simulink model "a_test"  (R2022b)
settings: Solver=VariableStepAuto  StartTime=0.0  StopTime=10.0  RelTol=1e-3
values from neighbouring files (symbols this model uses):
  L = 0.00046    [electric_current_loop.m]    (also in electric_kp_ki.m; pll.m = 10000; sl_ekf.m = c.L_LINE; sl_flux.m = L_avg - 0.5 * L_diff + L_diff * iq_obs * iq_obs / i2_obs)
undefined symbols (not defined in the file or in its folder): D_PI_I, D_PI_KB, D_PI_LOW_LIMIT, D_PI_P, D_PI_UP_LIMIT, Q_PI_I, Q_PI_KB, Q_PI_LOW_LIMIT, Q_PI_P, Q_PI_UP_LIMIT
libraries: slpidlib x6, spsPermanentMagnetSynchronousMachineLib x4, simulink x4, spsDCVoltageSourceLib x2, spsGroundLib x2, spsThreePhaseVIMeasurementLib x2, spsUniversalBridgeLib x2, spspowerguiLib x2
(part 1 of 2)
settings Model: Creator=15403  LastModifiedBy=15403

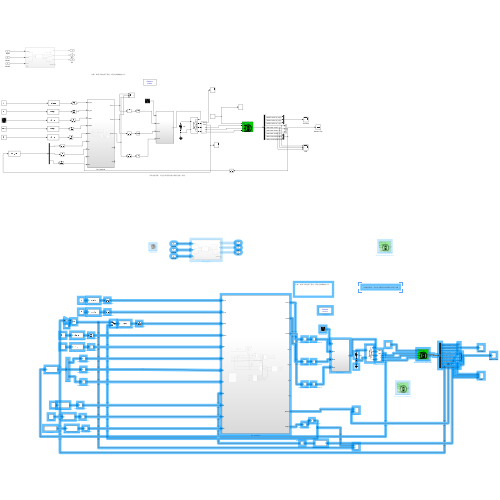
[thumbnail: Simulink's stored preview of the top-level diagram]
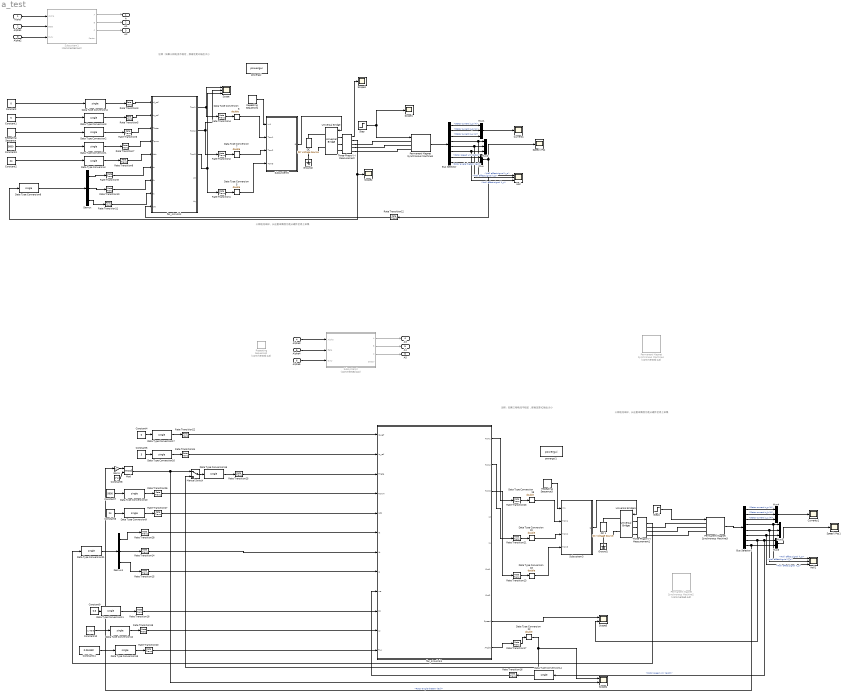
== system a_test ==
  note: 三相电流采样，从这里采集因为是从硬件全桥上采集
  note: 注释：如果三相电流不稳定，那肯定是IQ输出太小
  note: 注释：如果三相电流不稳定，那肯定是IQ输出太小
  note: 三相电流采样，从这里采集因为是从硬件全桥上采集
  Alpha : Inport
  Alpha1 : Inport  Port=2
  Alpha2 : Inport  Port=3
  Alpha3 : Inport  Port=4
  Alpha4 : Inport  Port=5
  Alpha5 : Inport  Port=6
  Bus Selector : BusSelector  OutputSignals=Stator current is_a (A),Stator current is_b (A),Stator current is_c (A),Hall effect signal h_a,Hall effect signal h_b,Hall effect signal h_c,Rotor speed wm (rad/s),Rotor angle thetam (rad)
  Bus Selector1 : BusSelector  OutputSignals=Stator current is_a (A),Stator current is_b (A),Stator current is_c (A),Hall effect signal h_a,Hall effect signal h_b,Hall effect signal h_c,Rotor speed wm (rad/s),Rotor angle thetam (rad)
  Constant : Constant  Value=0
  Constant1 : Constant  Value=5
  Constant10 : Constant  Value=1.4e-3
  Constant11 : Constant  Value=0.034182
  Constant2 : Constant  Value=24
  Constant3 : Constant  Value=5600
  Constant4 : Constant  Value=0
  Constant5 : Constant  Value=3
  Constant6 : Constant  Value=24
  Constant7 : Constant  Value=5600
  Constant8 : Constant  Value=2*pi
  Constant9 : Constant  Value=0.6
  Currents : Scope
  Currents1 : Scope
  "DC " : spsDCVoltageSourceLib/DC Voltage Source  Amplitude=24  Measurements=None
  DC 1 : spsDCVoltageSourceLib/DC Voltage Source  Amplitude=24  Measurements=None
  Data Type Conversion{,1..4,8..17,21} (16 alike) : DataTypeConversion  OutDataTypeStr=single  SaturateOnIntegerOverflow=off  RndMeth=Floor
  Data Type Conversion{5..7,18..20,22} (7 alike) : DataTypeConversion  OutDataTypeStr=double  SaturateOnIntegerOverflow=off  RndMeth=Floor
  Demux : Demux  Outputs=3
  Demux1 : Demux  Outputs=3
  Gain1 : Gain  OutDataTypeStr=double
  Ground1 : spsGroundLib/Ground  LConnTagsString=a
  Ground2 : spsGroundLib/Ground  LConnTagsString=a
  Hall : Scope  NumInputPorts=3
  Hall1 : Scope  NumInputPorts=3
  Manual Switch : ManualSwitch
  Mod : Math  Operator=mod  SignedPower=on
  Mux : Mux  Inputs=2
  Mux{1..2,4..5} (4 alike) : Mux  Inputs=3
  Mux3 : Mux  Inputs=2
  Permanent Magnet Synchronous Machine1 : spsPermanentMagnetSynchronousMachineLib/Permanent Magnet Synchronous Machine  NbPhases=3  FluxDistribution=Sinusoidal  RotorType=Round  MechanicalLoad=Torque Tm  PresetModel=No  ShowDetailedParameters=on  MeasurementBus=off  Resistance=0.6  Inductance=8.5e-3  dqInductances=[8.5e-3, 8.5e-3]  La=1.4e-3  MachineConstant=Flux linkage established by magnets (V.s)  Flux=0.034182  VoltageCst=6.1999  TorqueCst=0.051273  Flat=120  Mechanical=[1.1e-5,1e-4,1,0.02]  PolePairs=4  InitialConditions=[0,0, 0,0]  InitialConditions5ph=[0 0 0 0 0 0]  RefAngle=Aligned with phase A axis (original Park)  IterativeDiscreteModel=Trapezoidal non iterative  TsBlock=-1  TsPowergui=0
  Permanent Magnet Synchronous Machine2 : spsPermanentMagnetSynchronousMachineLib/Permanent Magnet Synchronous Machine  Commented=on  NbPhases=3  FluxDistribution=Sinusoidal  RotorType=Round  MechanicalLoad=Torque Tm  PresetModel=No  ShowDetailedParameters=on  MeasurementBus=off  Resistance=0.6  Inductance=8.5e-3  dqInductances=[8.5e-3, 8.5e-3]  La=1.4e-3  MachineConstant=Flux linkage established by magnets (V.s)  Flux=0.034182  VoltageCst=6.1999  TorqueCst=0.051273  Flat=120  Mechanical=[1.1e-5,1e-4,1,0.02]  PolePairs=4  InitialConditions=[0,0, 0,0]  InitialConditions5ph=[0 0 0 0 0 0]  RefAngle=Aligned with phase A axis (original Park)  IterativeDiscreteModel=Trapezoidal non iterative  TsBlock=-1  TsPowergui=0
  Permanent Magnet Synchronous Machine3 : spsPermanentMagnetSynchronousMachineLib/Permanent Magnet Synchronous Machine  NbPhases=3  FluxDistribution=Sinusoidal  RotorType=Round  MechanicalLoad=Torque Tm  PresetModel=No  ShowDetailedParameters=on  MeasurementBus=off  Resistance=0.6  Inductance=8.5e-3  dqInductances=[8.5e-3, 8.5e-3]  La=1.4e-3  MachineConstant=Flux linkage established by magnets (V.s)  Flux=0.034182  VoltageCst=6.1999  TorqueCst=0.051273  Flat=120  Mechanical=[1.1e-5,1e-4,1,0.02]  PolePairs=4  InitialConditions=[0,0, 0,0]  InitialConditions5ph=[0 0 0 0 0 0]  RefAngle=Aligned with phase A axis (original Park)  IterativeDiscreteModel=Trapezoidal non iterative  TsBlock=-1  TsPowergui=0
  Permanent Magnet Synchronous Machine4 : spsPermanentMagnetSynchronousMachineLib/Permanent Magnet Synchronous Machine  Commented=on  NbPhases=3  FluxDistribution=Sinusoidal  RotorType=Round  MechanicalLoad=Torque Tm  PresetModel=No  ShowDetailedParameters=on  MeasurementBus=off  Resistance=0.6  Inductance=8.5e-3  dqInductances=[8.5e-3, 8.5e-3]  La=1.4e-3  MachineConstant=Voltage Constant (V_peak L-L / krpm)  Flux=0.017643  VoltageCst=3.2  TorqueCst=0.026464  Flat=120  Mechanical=[1.1e-5,1e-4,1,0.02]  PolePairs=4  InitialConditions=[0,0, 0,0]  InitialConditions5ph=[0 0 0 0 0 0]  RefAngle=Aligned with phase A axis (original Park)  IterativeDiscreteModel=Trapezoidal non iterative  TsBlock=-1  TsPowergui=0
  Rate Transition{1..28} (28 alike) : RateTransition
  Repeating Sequence : simulink/Sources/Repeating Sequence  rep_seq_t=[0 0.1]  rep_seq_y=[0 2 * pi]
  Repeating Sequence1 : simulink/Sources/Repeating Sequence  rep_seq_t=[0 1/15000 2/15000]  rep_seq_y=[0 2800 0]
  Repeating Sequence2 : simulink/Sources/Repeating Sequence  Commented=on  rep_seq_t=[0 0.1]  rep_seq_y=[0 2 * pi]
  Repeating Sequence3 : simulink/Sources/Repeating Sequence  rep_seq_t=[0 1/15000 2/15000]  rep_seq_y=[0 2800 0]
  Scope : Scope  NumInputPorts=3
  Scope1 : Scope
  Scope2 : Scope
  Scope3 : Scope
  Scope4 : Scope  NumInputPorts=2
  Scope5 : Scope  NumInputPorts=2
  Speed / Pos : Scope
  Speed / Pos1 : Scope
  Step : Step  Time=0  After=0  SampleTime=0
  Step1 : Step  Time=0  After=0  SampleTime=0
  Subsystem1 : Subsystem  Commented=on
  Subsystem2 : Subsystem  Commented=on
  Subsystem3 : Subsystem
  Subsystem5 : Subsystem
  Three-Phase V-I Measurement : spsThreePhaseVIMeasurementLib/Three-Phase V-I Measurement  VoltageMeasurement=phase-to-ground  SetLabelV=off  LabelV=Vabc  Vpu=off  VpuLL=off  CurrentMeasurement=yes  SetLabelI=off  LabelI=Iabc  Ipu=off  Pbase=100e6  Vbase=500e3  OutputType=Complex  PhasorSimulation=off  PSBequivalent=0
  Three-Phase V-I Measurement1 : spsThreePhaseVIMeasurementLib/Three-Phase V-I Measurement  VoltageMeasurement=phase-to-ground  SetLabelV=off  LabelV=Vabc  Vpu=off  VpuLL=off  CurrentMeasurement=yes  SetLabelI=off  LabelI=Iabc  Ipu=off  Pbase=100e6  Vbase=500e3  OutputType=Complex  PhasorSimulation=off  PSBequivalent=0
  Universal Bridge : spsUniversalBridgeLib/Universal Bridge  Arms=3  SnubberResistance=1e5  SnubberCapacitance=inf  Device=IGBT / Diodes  Ron=1e-3  Lon=0  ForwardVoltages="[  0  0  ]"  ForwardVoltage=0  GTOparameters=[ 10e-6 , 20e-6 ]  IGBTparameters=[ 1e-6 , 2e-6 ]  Measurements=None  Measurements_2=None  converterType=Rectifier
  Universal Bridge1 : spsUniversalBridgeLib/Universal Bridge  Arms=3  SnubberResistance=1e5  SnubberCapacitance=inf  Device=IGBT / Diodes  Ron=1e-3  Lon=0  ForwardVoltages="[  0  0  ]"  ForwardVoltage=0  GTOparameters=[ 10e-6 , 20e-6 ]  IGBTparameters=[ 1e-6 , 2e-6 ]  Measurements=None  Measurements_2=None  converterType=Rectifier
  foc_simulink : Subsystem
  foc_simulink1 : Subsystem
  powergui : spspowerguiLib/powergui  Priority=1  SimulationMode=Discrete  SampleTime=0.000001  frequency=60  Iterations=50  frequencyindice=0  Pbase=100e6  ErrMax=1e-4  UnitsV=kV  UnitsW=MW  buscounter=0  FunctionMessages=off  echomessages=off  EnableUseOfTLC=off  CurrentSourceSwitches=off  DisableSnubberDevices=off  DisableRonSwitches=off  DisableVfSwitches=off  DisplayEquations=off  AutomaticDiscreteSolvers=off  SolverType=Tustin/Backward Euler (TBE)  Interpol=off  ExternalGateDelay=off  methode=off  Ts=100  x0status=blocks  SPID=on  SwTol=0  HookPort=off  NonlinearTolerance=1e-4  nMaxIteration=100  ContinueOnMaxIteration=off  RestoreLinks=warning  ResistiveCurrentMeasurement=off  Frange=[0:2:500]  Ylog=off  Xlog=on  ShowGrid=off  save=off  variable=ZData  structure=0  ZoomFFT=off  StartTime=0.0  cycles=1  DisplayStyle=1  fundamental=60  FreqAxis=off  MaxFrequency=1000  frequencyindicesteady=1  RmsSteady=1  display=off
  powergui1 : spspowerguiLib/powergui  Priority=1  SimulationMode=Discrete  SampleTime=0.000001  frequency=60  Iterations=50  frequencyindice=0  Pbase=100e6  ErrMax=1e-4  UnitsV=kV  UnitsW=MW  buscounter=0  FunctionMessages=off  echomessages=off  EnableUseOfTLC=off  CurrentSourceSwitches=off  DisableSnubberDevices=off  DisableRonSwitches=off  DisableVfSwitches=off  DisplayEquations=off  AutomaticDiscreteSolvers=off  SolverType=Tustin/Backward Euler (TBE)  Interpol=off  ExternalGateDelay=off  methode=off  Ts=100  x0status=blocks  SPID=on  SwTol=0  HookPort=off  NonlinearTolerance=1e-4  nMaxIteration=100  ContinueOnMaxIteration=off  RestoreLinks=warning  ResistiveCurrentMeasurement=off  Frange=[0:2:500]  Ylog=off  Xlog=on  ShowGrid=off  save=off  variable=ZData  structure=0  ZoomFFT=off  StartTime=0.0  cycles=1  DisplayStyle=1  fundamental=60  FreqAxis=off  MaxFrequency=1000  frequencyindicesteady=1  RmsSteady=1  display=off
  A : Outport
  A1 : Outport  Port=2
  A2 : Outport  Port=3
  A3 : Outport  Port=4
  A4 : Outport  Port=5
  A5 : Outport  Port=6
  wires:
  Data Type Conversion6/1 -> Subsystem5/2(Tcm1)
  Data Type Conversion8/1 -> Demux/1
  Rate Transition12/1 -> foc_simulink/9(we)
  Mux/1 -> Rate Transition12/1, Speed / Pos/1
  Three-Phase V-I Measurement/1 -> Scope3/1
  Demux/1 -> Rate Transition9/1
  Repeating Sequence/1 -> Data Type Conversion2/1
  Constant/1 -> Data Type Conversion4/1
  Alpha/1 -> Subsystem1/1(Alpha)
  Bus Selector/4 -> Hall/1, Mux2/1  "<Hall effect signal h_a>"
  Subsystem1/3(C) -> A2/1
  Data Type Conversion7/1 -> Subsystem5/3(Tcm2)
  Alpha2/1 -> Subsystem1/3(Duty)
  Data Type Conversion5/1 -> Subsystem5/4(Tcm3)
  Subsystem1/1(A) -> A/1
  Rate Transition6/1 -> foc_simulink/3(Theta)
  Data Type Conversion/1 -> Rate Transition8/1
  Rate Transition9/1 -> foc_simulink/6(Ia)
  Demux/2 -> Rate Transition10/1
  Rate Transition11/1 -> foc_simulink/8(Ic)
  Data Type Conversion1/1 -> Rate Transition7/1
  Subsystem1/2(B) -> A1/1
  Constant3/1 -> Data Type Conversion1/1
  Demux/3 -> Rate Transition11/1
  Rate Transition1/1 -> Data Type Conversion5/1
  Rate Transition10/1 -> foc_simulink/7(Ib)
  Repeating Sequence1/1 -> Subsystem5/1(In1)
  Subsystem5/1(g) -> Universal Bridge/1
  Rate Transition8/1 -> foc_simulink/5(Udc)
  Rate Transition4/1 -> Data Type Conversion6/1
  Rate Transition5/1 -> foc_simulink/2(Iq_ref)
  Constant1/1 -> Data Type Conversion3/1
  Rate Transition2/1 -> Data Type Conversion7/1
  Permanent Magnet Synchronous Machine1/1 -> Bus Selector/1
  Data Type Conversion2/1 -> Rate Transition6/1
  Step/1 -> Permanent Magnet Synchronous Machine1/1, Scope1/1
  Mux1/1 -> Currents/1
  Bus Selector/6 -> Mux2/3, Hall/3  "<Hall effect signal h_c>"
  Bus Selector/1 -> Mux1/1  "<Stator current is_a (A)>"
  Rate Transition3/1 -> foc_simulink/1(Id_ref)
  Data Type Conversion3/1 -> Rate Transition5/1
  Bus Selector/3 -> Mux1/3  "<Stator current is_c (A)>"
  Constant2/1 -> Data Type Conversion/1
  Bus Selector/8 -> Mux/2  "<Rotor angle thetam (rad)>"
  Bus Selector/5 -> Mux2/2, Hall/2  "<Hall effect signal h_b>"
  Rate Transition7/1 -> foc_simulink/4(Tpwm)
  foc_simulink/2(Tcm2) -> Rate Transition2/1, Scope/2
  Three-Phase V-I Measurement/2 -> Scope2/1, Data Type Conversion8/1
  Data Type Conversion4/1 -> Rate Transition3/1
  foc_simulink/1(Tcm1) -> Rate Transition4/1, Scope/1
  Bus Selector/7 -> Mux/1  "<Rotor speed wm (rad/s)>"
  foc_simulink/3(Tcm3) -> Rate Transition1/1, Scope/3
  Bus Selector/2 -> Mux1/2  "<Stator current is_b (A)>"
  Alpha1/1 -> Subsystem1/2(Beta)
  Data Type Conversion14/1 -> Rate Transition16/1
  Mod/1 -> Scope4/2, Manual Switch/1
  Data Type Conversion18/1 -> Subsystem3/4(Tcm3)
  foc_simulink1/8(Speed) -> Scope5/1
  foc_simulink1/3(Tcm3) -> Rate Transition13/1
  Permanent Magnet Synchronous Machine3/1 -> Bus Selector1/1
  foc_simulink1/9(Angle) -> Rate Transition17/1
  Rate Transition19/1 -> foc_simulink1/11(Ls)
  Constant11/1 -> Data Type Conversion13/1
  Data Type Conversion13/1 -> Rate Transition20/1
  Gain1/1 -> Mod/1
  Rate Transition28/1 -> foc_simulink1/6(Ia)
  Alpha4/1 -> Subsystem2/2(Beta)
  Rate Transition18/1 -> foc_simulink1/10(Rs)
  Data Type Conversion16/1 -> Rate Transition24/1
  Rate Transition21/1 -> Data Type Conversion20/1
  Rate Transition20/1 -> foc_simulink1/12(flux)
  Bus Selector1/7 -> Scope5/2, Data Type Conversion14/1, Mux3/1  "<Rotor speed wm (rad/s)>"
  Bus Selector1/5 -> Mux5/2, Hall1/2  "<Hall effect signal h_b>"
  Subsystem2/3(C) -> A5/1
  Data Type Conversion15/1 -> Rate Transition25/1
  Bus Selector1/2 -> Mux4/2  "<Stator current is_b (A)>"
  Data Type Conversion11/1 -> Rate Transition18/1
  Manual Switch/1 -> Data Type Conversion15/1
  Step1/1 -> Permanent Magnet Synchronous Machine3/1
  Subsystem3/1(g) -> Universal Bridge1/1
  Bus Selector1/3 -> Mux4/3  "<Stator current is_c (A)>"
  Data Type Conversion22/1 -> Scope4/1, Manual Switch/2
  Three-Phase V-I Measurement1/2 -> Data Type Conversion21/1
  foc_simulink1/1(Tcm1) -> Rate Transition23/1
  foc_simulink1/2(Tcm2) -> Rate Transition21/1
  Rate Transition26/1 -> foc_simulink1/4(Tpwm)
  Constant9/1 -> Data Type Conversion11/1
  Constant5/1 -> Data Type Conversion16/1
  Bus Selector1/6 -> Mux5/3, Hall1/3  "<Hall effect signal h_c>"
  Constant8/1 -> Mod/2
  Constant6/1 -> Data Type Conversion9/1
  Bus Selector1/8 -> Mux3/2, Gain1/1  "<Rotor angle thetam (rad)>"
  Bus Selector1/1 -> Mux4/1  "<Stator current is_a (A)>"
  Rate Transition27/1 -> foc_simulink1/5(Udc)
  Subsystem2/1(A) -> A3/1
  Rate Transition22/1 -> foc_simulink1/1(Id_ref)
  Bus Selector1/4 -> Hall1/1, Mux5/1  "<Hall effect signal h_a>"
  Mux4/1 -> Currents1/1
  Demux1/1 -> Rate Transition28/1
  Data Type Conversion21/1 -> Demux1/1
  Rate Transition24/1 -> foc_simulink1/2(Iq_ref)
  Repeating Sequence3/1 -> Subsystem3/1(In1)
  Rate Transition25/1 -> foc_simulink1/3(Theta)
  Alpha3/1 -> Subsystem2/1(Alpha)
  Demux1/3 -> Rate Transition15/1
  Demux1/2 -> Rate Transition14/1
  Data Type Conversion20/1 -> Subsystem3/3(Tcm2)
  Constant4/1 -> Data Type Conversion17/1
  Constant7/1 -> Data Type Conversion10/1
  Rate Transition13/1 -> Data Type Conversion18/1
  Mux3/1 -> Speed / Pos1/1
  Constant10/1 -> Data Type Conversion12/1
  Subsystem2/2(B) -> A4/1
  Rate Transition17/1 -> Data Type Conversion22/1
  Rate Transition15/1 -> foc_simulink1/8(Ic)
  Data Type Conversion17/1 -> Rate Transition22/1
  Data Type Conversion10/1 -> Rate Transition26/1
  Data Type Conversion9/1 -> Rate Transition27/1
  Alpha5/1 -> Subsystem2/3(Duty)
  Rate Transition14/1 -> foc_simulink1/7(Ib)
  Data Type Conversion12/1 -> Rate Transition19/1
  Rate Transition23/1 -> Data Type Conversion19/1
  Rate Transition16/1 -> foc_simulink1/9(we)
  Data Type Conversion19/1 -> Subsystem3/2(Tcm1)
  connections:
  Ground2/LConn1 -- "DC "/LConn1 -- Universal Bridge/RConn2
  "DC "/RConn1 -- Universal Bridge/RConn1
  Universal Bridge/LConn2 -- Three-Phase V-I Measurement/LConn2
  Three-Phase V-I Measurement/RConn3 -- Permanent Magnet Synchronous Machine1/LConn3
  Universal Bridge/LConn3 -- Three-Phase V-I Measurement/LConn3
  Three-Phase V-I Measurement/RConn2 -- Permanent Magnet Synchronous Machine1/LConn2
  Universal Bridge/LConn1 -- Three-Phase V-I Measurement/LConn1
  Three-Phase V-I Measurement/RConn1 -- Permanent Magnet Synchronous Machine1/LConn1
  Universal Bridge1/RConn2 -- Ground1/LConn1 -- DC 1/LConn1
  Universal Bridge1/LConn2 -- Three-Phase V-I Measurement1/LConn2
  Permanent Magnet Synchronous Machine3/LConn2 -- Three-Phase V-I Measurement1/RConn2
  Universal Bridge1/LConn1 -- Three-Phase V-I Measurement1/LConn1
  DC 1/RConn1 -- Universal Bridge1/RConn1
  Universal Bridge1/LConn3 -- Three-Phase V-I Measurement1/LConn3
  Permanent Magnet Synchronous Machine3/LConn3 -- Three-Phase V-I Measurement1/RConn3
  Permanent Magnet Synchronous Machine3/LConn1 -- Three-Phase V-I Measurement1/RConn1

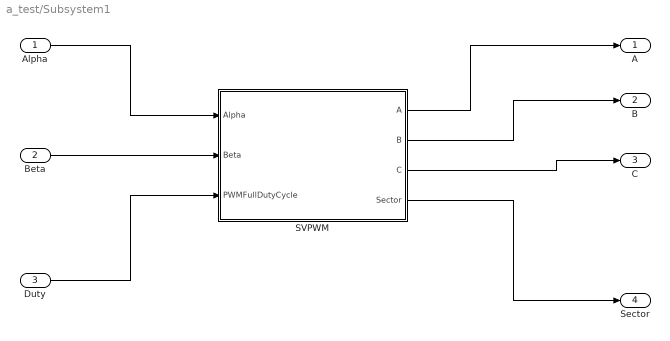
== system a_test/Subsystem1 ==
  Alpha : Inport
  Beta : Inport  Port=2
  Duty : Inport  Port=3
  SVPWM : MATLAB Function  TreatAsAtomicUnit=on
  A : Outport
  B : Outport  Port=2
  C : Outport  Port=3
  Sector : Outport  Port=4
  wires:
  SVPWM/1(A) -> A/1
  Duty/1 -> SVPWM/3(PWMFullDutyCycle)
  Alpha/1 -> SVPWM/1(Alpha)
  Beta/1 -> SVPWM/2(Beta)
  SVPWM/3(C) -> C/1
  SVPWM/4(Sector) -> Sector/1
  SVPWM/2(B) -> B/1

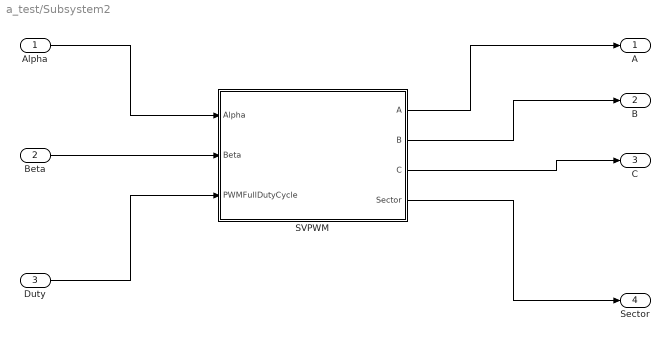
== system a_test/Subsystem2 ==
  Alpha : Inport
  Beta : Inport  Port=2
  Duty : Inport  Port=3
  SVPWM : MATLAB Function  TreatAsAtomicUnit=on
  A : Outport
  B : Outport  Port=2
  C : Outport  Port=3
  Sector : Outport  Port=4
  wires:
  SVPWM/1(A) -> A/1
  Duty/1 -> SVPWM/3(PWMFullDutyCycle)
  Alpha/1 -> SVPWM/1(Alpha)
  Beta/1 -> SVPWM/2(Beta)
  SVPWM/3(C) -> C/1
  SVPWM/4(Sector) -> Sector/1
  SVPWM/2(B) -> B/1

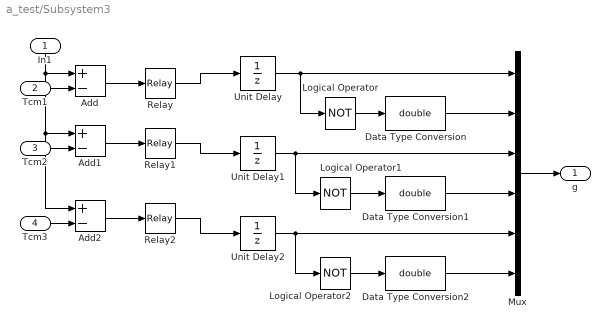
== system a_test/Subsystem3 ==
  In1 : Inport
  Tcm1 : Inport  Port=2
  Tcm2 : Inport  Port=3
  Tcm3 : Inport  Port=4
  Add : Sum  Inputs=+-
  Add1 : Sum  Inputs=+-
  Add2 : Sum  Inputs=+-
  Data Type Conversion : DataTypeConversion  OutDataTypeStr=double  SaturateOnIntegerOverflow=off  RndMeth=Floor
  Data Type Conversion1 : DataTypeConversion  OutDataTypeStr=double  SaturateOnIntegerOverflow=off  RndMeth=Floor
  Data Type Conversion2 : DataTypeConversion  OutDataTypeStr=double  SaturateOnIntegerOverflow=off  RndMeth=Floor
  Logical Operator : Logic  Operator=NOT  AllPortsSameDT=off  OutDataTypeStr=boolean
  Logical Operator1 : Logic  Operator=NOT  AllPortsSameDT=off  OutDataTypeStr=boolean
  Logical Operator2 : Logic  Operator=NOT  AllPortsSameDT=off  OutDataTypeStr=boolean
  Mux : Mux  Inputs=6
  Relay : Relay  OffSwitchValue=-eps
  Relay1 : Relay  OffSwitchValue=-eps
  Relay2 : Relay  OffSwitchValue=-eps
  Unit Delay : UnitDelay  SampleTime=-1  HasFrameUpgradeWarning=on
  Unit Delay1 : UnitDelay  SampleTime=-1  HasFrameUpgradeWarning=on
  Unit Delay2 : UnitDelay  SampleTime=-1  HasFrameUpgradeWarning=on
  g : Outport  VectorParamsAs1DForOutWhenUnconnected=off
  wires:
  Tcm3/1 -> Add2/2
  Tcm2/1 -> Add1/2
  Tcm1/1 -> Add/2
  Relay2/1 -> Unit Delay2/1
  Relay1/1 -> Unit Delay1/1
  Relay/1 -> Unit Delay/1
  Unit Delay2/1 -> Mux/5, Logical Operator2/1
  Unit Delay1/1 -> Mux/3, Logical Operator1/1
  Unit Delay/1 -> Logical Operator/1, Mux/1
  Mux/1 -> g/1
  Data Type Conversion/1 -> Mux/2
  Data Type Conversion1/1 -> Mux/4
  Data Type Conversion2/1 -> Mux/6
  Logical Operator2/1 -> Data Type Conversion2/1
  Logical Operator1/1 -> Data Type Conversion1/1
  Logical Operator/1 -> Data Type Conversion/1
  Add1/1 -> Relay1/1
  Add2/1 -> Relay2/1
  Add/1 -> Relay/1
  In1/1 -> Add/1, Add2/1, Add1/1

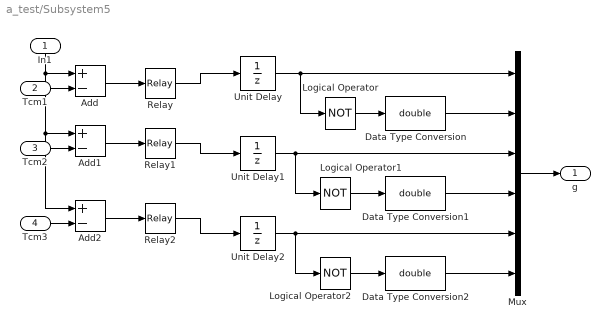
== system a_test/Subsystem5 ==
  In1 : Inport
  Tcm1 : Inport  Port=2
  Tcm2 : Inport  Port=3
  Tcm3 : Inport  Port=4
  Add : Sum  Inputs=+-
  Add1 : Sum  Inputs=+-
  Add2 : Sum  Inputs=+-
  Data Type Conversion : DataTypeConversion  OutDataTypeStr=double  SaturateOnIntegerOverflow=off  RndMeth=Floor
  Data Type Conversion1 : DataTypeConversion  OutDataTypeStr=double  SaturateOnIntegerOverflow=off  RndMeth=Floor
  Data Type Conversion2 : DataTypeConversion  OutDataTypeStr=double  SaturateOnIntegerOverflow=off  RndMeth=Floor
  Logical Operator : Logic  Operator=NOT  AllPortsSameDT=off  OutDataTypeStr=boolean
  Logical Operator1 : Logic  Operator=NOT  AllPortsSameDT=off  OutDataTypeStr=boolean
  Logical Operator2 : Logic  Operator=NOT  AllPortsSameDT=off  OutDataTypeStr=boolean
  Mux : Mux  Inputs=6
  Relay : Relay  OffSwitchValue=-eps
  Relay1 : Relay  OffSwitchValue=-eps
  Relay2 : Relay  OffSwitchValue=-eps
  Unit Delay : UnitDelay  SampleTime=-1  HasFrameUpgradeWarning=on
  Unit Delay1 : UnitDelay  SampleTime=-1  HasFrameUpgradeWarning=on
  Unit Delay2 : UnitDelay  SampleTime=-1  HasFrameUpgradeWarning=on
  g : Outport  VectorParamsAs1DForOutWhenUnconnected=off
  wires:
  Tcm3/1 -> Add2/2
  Tcm2/1 -> Add1/2
  Tcm1/1 -> Add/2
  Relay2/1 -> Unit Delay2/1
  Relay1/1 -> Unit Delay1/1
  Relay/1 -> Unit Delay/1
  Unit Delay2/1 -> Mux/5, Logical Operator2/1
  Unit Delay1/1 -> Mux/3, Logical Operator1/1
  Unit Delay/1 -> Logical Operator/1, Mux/1
  Mux/1 -> g/1
  Data Type Conversion/1 -> Mux/2
  Data Type Conversion1/1 -> Mux/4
  Data Type Conversion2/1 -> Mux/6
  Logical Operator2/1 -> Data Type Conversion2/1
  Logical Operator1/1 -> Data Type Conversion1/1
  Logical Operator/1 -> Data Type Conversion/1
  Add1/1 -> Relay1/1
  Add2/1 -> Relay2/1
  Add/1 -> Relay/1
  In1/1 -> Add/1, Add2/1, Add1/1

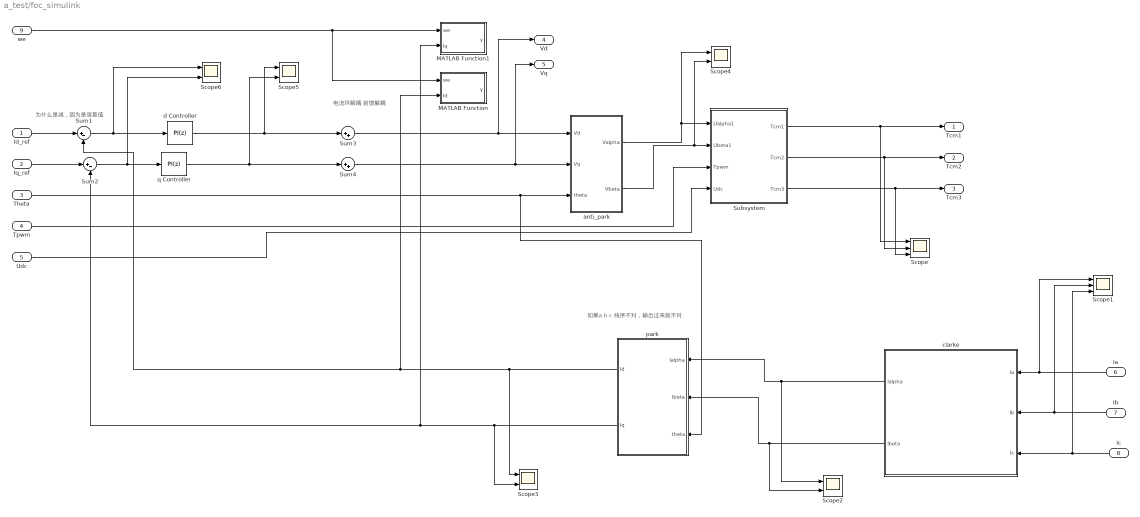
== system a_test/foc_simulink ==
  note: 电流环解耦
      | 前馈解耦
  note: 为什么是减，因为是误差值
  note: 如果a b c 线序不对，输出过来就不对
  Id_ref : Inport
  Iq_ref : Inport  Port=2
  Theta : Inport  Port=3
  Tpwm : Inport  Port=4
  Udc : Inport  Port=5
  Ia : Inport  Port=6
  Ib : Inport  Port=7
  Ic : Inport  Port=8
  we : Inport  Port=9
  MATLAB Function : MATLAB Function  TreatAsAtomicUnit=on
  MATLAB Function1 : MATLAB Function  TreatAsAtomicUnit=on
  Scope : Scope  NumInputPorts=3
  Scope1 : Scope  NumInputPorts=3
  Scope{2..6} (5 alike) : Scope  NumInputPorts=2
  Subsystem : Subsystem
  Sum1 : Sum  Inputs=|+-
  Sum2 : Sum  Inputs=|+-
  Sum3 : Sum  Inputs=|++  AccumDataTypeStr=single  OutDataTypeStr=single
  Sum4 : Sum  Inputs=|++  AccumDataTypeStr=single  OutDataTypeStr=single
  anti_park : Subsystem
  clarke : Subsystem
  d Controller : slpidlib/PID Controller  Controller=PI  Form=Parallel  TimeDomain=Discrete-time  UseExternalTs=off  SampleTime=-1  IntegratorMethod=Forward Euler  FilterMethod=Forward Euler  ControllerParametersSource=internal  P=D_PI_P  I=D_PI_I  UseKiTs=off  D=0.09  N=100  UseFilter=on  TunerSelectOption=Transfer Function Based (PID Tuner App)  InitialConditionSource=internal  InitialConditionForIntegrator=0  InitialConditionForFilter=0  DifferentiatorICPrevScaledInput=0  ExternalReset=none  TrackingMode=off  Kt=1  LimitOutput=on  SatLimitsSource=internal  UpperSaturationLimit=D_PI_UP_LIMIT  LowerSaturationLimit=D_PI_LOW_LIMIT  LinearizeAsGain=off  AntiWindupMode=back-calculation  Kb=D_PI_KB  LimitIntegrator=off  UpperIntegratorSaturationLimit=inf  LowerIntegratorSaturationLimit=-inf  PGainOutDataTypeStr=single  PProdOutDataTypeStr=single  POutMin=[]  POutMax=[]  IGainOutDataTypeStr=single  IProdOutDataTypeStr=single  IOutMin=[]  IOutMax=[]  DOutMin=[]  DOutMax=[]  NOutMin=[]  NOutMax=[]  SumOutDataTypeStr=single  SumOutMin=[]  SumOutMax=[]  SaturationOutDataTypeStr=single  SaturationOutMin=[]  SaturationOutMax=[]  PParamDataTypeStr=single  PParamMin=[]  PParamMax=[]  IParamDataTypeStr=single  IParamMin=[]  IParamMax=[]  DParamMin=[]  DParamMax=[]  NParamMin=[]  NParamMax=[]  KbParamDataTypeStr=single  KbParamMin=[]  KbParamMax=[]  KtParamMin=[]  KtParamMax=[]  KbOutDataTypeStr=single  KbOutMin=[]  KbOutMax=[]  KtOutMin=[]  KtOutMax=[]  IntegratorOutDataTypeStr=single  IntegratorOutMin=[]  IntegratorOutMax=[]  FilterOutMin=[]  FilterOutMax=[]  SumI1OutDataTypeStr=single  SumI1OutMin=[]  SumI1OutMax=[]  SumI2OutDataTypeStr=single  SumI2OutMin=[]  SumI2OutMax=[]  SumI3OutMin=[]  SumI3OutMax=[]  SumI4OutMin=[]  SumI4OutMax=[]  SumDOutMin=[]  SumDOutMax=[]  SumAccumDataTypeStr=single  SumI1AccumDataTypeStr=single  SumI2AccumDataTypeStr=single  DifferentiatorOutMin=[]  DifferentiatorOutMax=[]  FilterDiffOutCoefMin=[]  FilterDiffOutCoefMax=[]  ReciprocalOutMin=[]  ReciprocalOutMax=[]  SumDenOutMin=[]  SumDenOutMax=[]  SumNumOutMin=[]  SumNumOutMax=[]  DivideOutMin=[]  DivideOutMax=[]  UdiffTsProdOutMin=[]  UdiffTsProdOutMax=[]  NTsProdOutMin=[]  NTsProdOutMax=[]  UintegralTsProdOutMin=[]  UintegralTsProdOutMax=[]  UngainTsProdOutMin=[]  UngainTsProdOutMax=[]  ClampingZeroOutDataTypeStr=Inherit: Inherit via back propagation  ClampingZeroOutMin=[]  ClampingZeroOutMax=[]  FilterDenConstantOutDataTypeStr=Inherit: Inherit via back propagation  FilterDenConstantOutMin=[]  FilterDenConstantOutMax=[]  PCopyOutDataTypeStr=Inherit: Inherit via back propagation  PCopyOutMin=[]  PCopyOutMax=[]  NCopyOutDataTypeStr=Inherit: Inherit via back propagation  NCopyOutMin=[]  NCopyOutMax=[]  IntegratorContinuousStateAttributes=''  IntegratorStateIdentifier=di  IntegratorStateMustResolveToSignalObject=off  IntegratorRTWStateStorageClass=Auto  FilterContinuousStateAttributes=''  FilterStateMustResolveToSignalObject=off  FilterRTWStateStorageClass=Auto  ParallelPVariant=InternalParameters  IdealPVariant=Disabled  IVariant=InternalParameters  DVariant=Disabled  IntegratorVariant=Discrete  SatVariant=Enabled  AWVariant=BackCalculation  PCopyVariant=Disabled  TRVariant=Disabled  FdbkBlocksVariant=Forward  IdealPFdbkVariant=Disabled  SatFdbkVariant=Disabled  DerivativeFilterVariant=Disabled  NVariant=Disabled  NCopyVariant=Disabled_SignalSpec  FilterICVariant=Disabled  IntegratorICVariant=InternalICs  ExternalResetVariant=Disabled  TRSumVariant=Passthrough  SumFdbkVariant=Disabled  SumVariant=Sum_PI  TsampFilterVariant=InternalTs  TsampNgainVariant=Passthrough  TsampIntegralVariant=Passthrough  ExternalSaturationOutDataTypeStr=Inherit: Same as second input
  park : Subsystem
  q Controller : slpidlib/PID Controller  Controller=PI  Form=Parallel  TimeDomain=Discrete-time  UseExternalTs=off  SampleTime=-1  IntegratorMethod=Forward Euler  FilterMethod=Forward Euler  ControllerParametersSource=internal  P=Q_PI_P  I=Q_PI_I  UseKiTs=off  D=0.09  N=100  UseFilter=on  TunerSelectOption=Transfer Function Based (PID Tuner App)  InitialConditionSource=internal  InitialConditionForIntegrator=0  InitialConditionForFilter=0  DifferentiatorICPrevScaledInput=0  ExternalReset=none  TrackingMode=off  Kt=1  LimitOutput=on  SatLimitsSource=internal  UpperSaturationLimit=Q_PI_UP_LIMIT  LowerSaturationLimit=Q_PI_LOW_LIMIT  LinearizeAsGain=off  AntiWindupMode=back-calculation  Kb=Q_PI_KB  LimitIntegrator=off  UpperIntegratorSaturationLimit=inf  LowerIntegratorSaturationLimit=-inf  PGainOutDataTypeStr=single  PProdOutDataTypeStr=single  POutMin=[]  POutMax=[]  IGainOutDataTypeStr=single  IProdOutDataTypeStr=single  IOutMin=[]  IOutMax=[]  DOutMin=[]  DOutMax=[]  NOutMin=[]  NOutMax=[]  SumOutDataTypeStr=single  SumOutMin=[]  SumOutMax=[]  SaturationOutDataTypeStr=single  SaturationOutMin=[]  SaturationOutMax=[]  PParamDataTypeStr=single  PParamMin=[]  PParamMax=[]  IParamDataTypeStr=single  IParamMin=[]  IParamMax=[]  DParamMin=[]  DParamMax=[]  NParamMin=[]  NParamMax=[]  KbParamDataTypeStr=single  KbParamMin=[]  KbParamMax=[]  KtParamMin=[]  KtParamMax=[]  KbOutDataTypeStr=single  KbOutMin=[]  KbOutMax=[]  KtOutMin=[]  KtOutMax=[]  IntegratorOutDataTypeStr=single  IntegratorOutMin=[]  IntegratorOutMax=[]  FilterOutMin=[]  FilterOutMax=[]  SumI1OutDataTypeStr=single  SumI1OutMin=[]  SumI1OutMax=[]  SumI2OutDataTypeStr=single  SumI2OutMin=[]  SumI2OutMax=[]  SumI3OutMin=[]  SumI3OutMax=[]  SumI4OutMin=[]  SumI4OutMax=[]  SumDOutMin=[]  SumDOutMax=[]  SumAccumDataTypeStr=single  SumI1AccumDataTypeStr=single  SumI2AccumDataTypeStr=single  DifferentiatorOutMin=[]  DifferentiatorOutMax=[]  FilterDiffOutCoefMin=[]  FilterDiffOutCoefMax=[]  ReciprocalOutMin=[]  ReciprocalOutMax=[]  SumDenOutMin=[]  SumDenOutMax=[]  SumNumOutMin=[]  SumNumOutMax=[]  DivideOutMin=[]  DivideOutMax=[]  UdiffTsProdOutMin=[]  UdiffTsProdOutMax=[]  NTsProdOutMin=[]  NTsProdOutMax=[]  UintegralTsProdOutMin=[]  UintegralTsProdOutMax=[]  UngainTsProdOutMin=[]  UngainTsProdOutMax=[]  ClampingZeroOutDataTypeStr=Inherit: Inherit via back propagation  ClampingZeroOutMin=[]  ClampingZeroOutMax=[]  FilterDenConstantOutDataTypeStr=Inherit: Inherit via back propagation  FilterDenConstantOutMin=[]  FilterDenConstantOutMax=[]  PCopyOutDataTypeStr=Inherit: Inherit via back propagation  PCopyOutMin=[]  PCopyOutMax=[]  NCopyOutDataTypeStr=Inherit: Inherit via back propagation  NCopyOutMin=[]  NCopyOutMax=[]  IntegratorContinuousStateAttributes=''  IntegratorStateIdentifier=qi  IntegratorStateMustResolveToSignalObject=off  IntegratorRTWStateStorageClass=Auto  FilterContinuousStateAttributes=''  FilterStateMustResolveToSignalObject=off  FilterRTWStateStorageClass=Auto  ParallelPVariant=InternalParameters  IdealPVariant=Disabled  IVariant=InternalParameters  DVariant=Disabled  IntegratorVariant=Discrete  SatVariant=Enabled  AWVariant=BackCalculation  PCopyVariant=Disabled  TRVariant=Disabled  FdbkBlocksVariant=Forward  IdealPFdbkVariant=Disabled  SatFdbkVariant=Disabled  DerivativeFilterVariant=Disabled  NVariant=Disabled  NCopyVariant=Disabled_SignalSpec  FilterICVariant=Disabled  IntegratorICVariant=InternalICs  ExternalResetVariant=Disabled  TRSumVariant=Passthrough  SumFdbkVariant=Disabled  SumVariant=Sum_PI  TsampFilterVariant=InternalTs  TsampNgainVariant=Passthrough  TsampIntegralVariant=Passthrough  ExternalSaturationOutDataTypeStr=Inherit: Same as second input
  Tcm1 : Outport
  Tcm2 : Outport  Port=2
  Tcm3 : Outport  Port=3
  Vd : Outport  Port=4
  Vq : Outport  Port=5
  wires:
  Theta/1 -> anti_park/3(theta), park/3(theta)
  Udc/1 -> Subsystem/4(Udc)
  Tpwm/1 -> Subsystem/3(Tpwm)
  Subsystem/3(Tcm3) -> Scope/3, Tcm3/1
  anti_park/2(Vbeta) -> Scope4/2, Subsystem/2(Ubeta1)
  Subsystem/1(Tcm1) -> Scope/1, Tcm1/1
  Subsystem/2(Tcm2) -> Scope/2, Tcm2/1
  anti_park/1(Valpha) -> Scope4/1, Subsystem/1(Ualpha1)
  clarke/2(Ibeta) -> Scope2/2, park/2(Ibeta)
  clarke/1(Ialpha) -> Scope2/1, park/1(Ialpha)
  Ia/1 -> Scope1/1, clarke/1(Ia)
  Ib/1 -> Scope1/2, clarke/2(Ib)
  Ic/1 -> Scope1/3, clarke/3(Ic)
  park/1(Id) -> MATLAB Function/2(Id), Sum1/2, Scope3/1
  park/2(Iq) -> Scope3/2, Sum2/2, MATLAB Function1/2(Iq)
  Id_ref/1 -> Sum1/1
  Sum1/1 -> Scope6/1, d Controller/1
  Iq_ref/1 -> Sum2/1
  Sum2/1 -> Scope6/2, q Controller/1
  d Controller/1 -> Scope5/1, Sum3/1
  q Controller/1 -> Scope5/2, Sum4/1
  we/1 -> MATLAB Function/1(we), MATLAB Function1/1(we)
  Sum4/1 -> Vq/1, anti_park/2(Vq)
  Sum3/1 -> Vd/1, anti_park/1(Vd)

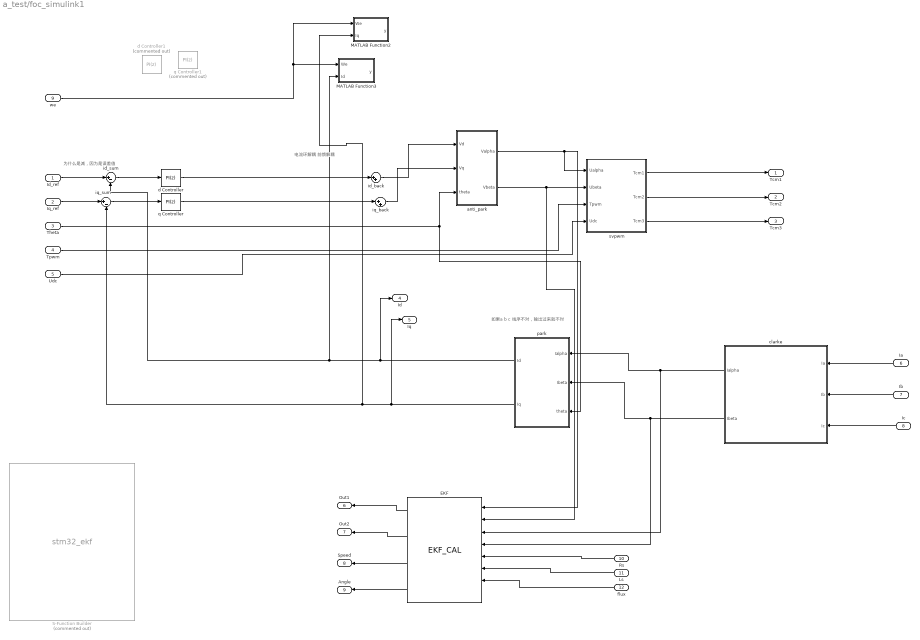
== system a_test/foc_simulink1 ==
  note: 电流环解耦
      | 前馈解耦
  note: 为什么是减，因为是误差值
  note: 如果a b c 线序不对，输出过来就不对
  Id_ref : Inport
  Iq_ref : Inport  Port=2
  Theta : Inport  Port=3
  Tpwm : Inport  Port=4
  Udc : Inport  Port=5
  Ia : Inport  Port=6
  Ib : Inport  Port=7
  Ic : Inport  Port=8
  we : Inport  Port=9
  Rs : Inport  Port=10
  Ls : Inport  Port=11
  flux : Inport  Port=12
  EKF : S-Function  FunctionName=EKF_CAL  SFunctionDeploymentMode=off  EnableBusSupport=off  mask(S-Function Builder){}
      mask help: Simulink:masks:SFunctionBuilder_MD
      mask init:
      | val = [[.9  0.75 0.75 1 1 .9 .9 1]',[1 1 0.75 0.75 .9 .9 1 .9]'];try , sys = get_param(gcb,'SfunBuilderFcnName');if isempty(sys), sys = get_param(gcb,'FunctionName'); end,catch, sys = get_param(gcb,'FunctionName'); end
      settings: CopyFcn=set_param(gcbh,'LinkStatus','none')  OpenFcn=sfunctionwizard(gcbh)
      mask Display: plot(val(:,1),val(:,2)),disp(sys),port_label('input',1,'Ualpha'),port_label('input',2,'Ubeta'),port_label('input',3,'Ialpha'),port_label('input',4,'Ibeta'),port_label('input',5,'Rs_in'),port_label('input',6,'Flux_in'),port_label('input',7,'Ls_in'),port_label('output',1,'y0'),port_label('output',2,'y1'),port_label('output',3,'Speed'),port_label('output',4,'Angle')
  MATLAB Function2 : MATLAB Function  TreatAsAtomicUnit=on
  MATLAB Function3 : MATLAB Function  TreatAsAtomicUnit=on
  S-Function Builder : S-Function  Commented=on  InitFcn=try, set_param(gcb,'FunctionName','stm32_ekf'), end  FunctionName=stm32_ekf  SFunctionModules=stm32_ekf_wrapper  SFunctionDeploymentMode=off  EnableBusSupport=off  mask(S-Function Builder){}
      mask help: Simulink:masks:SFunctionBuilder_MD
      mask init: same as a_test/foc_simulink1/EKF
      settings: CopyFcn=set_param(gcbh,'LinkStatus','none')  PreSaveFcn=try, set_param(gcb,'FunctionName','stm32_ekf'), end  OpenFcn=sfunctionwizard(gcbh)
      mask Display: plot(val(:,1),val(:,2)),disp(sys),port_label('input',1,'Ualpha'),port_label('input',2,'Ubeta'),port_label('input',3,'Ialpha'),port_label('input',4,'Ibeta'),port_label('input',5,'Rs_in'),port_label('input',6,'Ls_in'),port_label('input',7,'Flux_in'),port_label('input',8,'u0'),port_label('output',1,'y')
  anti_park : Subsystem
  clarke : Subsystem
  d Controller : slpidlib/PID Controller  Controller=PI  Form=Parallel  TimeDomain=Discrete-time  UseExternalTs=off  SampleTime=-1  IntegratorMethod=Forward Euler  FilterMethod=Forward Euler  ControllerParametersSource=internal  P=D_PI_P  I=D_PI_I  UseKiTs=off  D=0.09  N=100  UseFilter=on  TunerSelectOption=Transfer Function Based (PID Tuner App)  InitialConditionSource=internal  InitialConditionForIntegrator=0  InitialConditionForFilter=0  DifferentiatorICPrevScaledInput=0  ExternalReset=none  TrackingMode=off  Kt=1  LimitOutput=on  SatLimitsSource=internal  UpperSaturationLimit=D_PI_UP_LIMIT  LowerSaturationLimit=D_PI_LOW_LIMIT  LinearizeAsGain=off  AntiWindupMode=back-calculation  Kb=D_PI_KB  LimitIntegrator=off  UpperIntegratorSaturationLimit=inf  LowerIntegratorSaturationLimit=-inf  PGainOutDataTypeStr=single  PProdOutDataTypeStr=single  POutMin=[]  POutMax=[]  IGainOutDataTypeStr=single  IProdOutDataTypeStr=single  IOutMin=[]  IOutMax=[]  DOutMin=[]  DOutMax=[]  NOutMin=[]  NOutMax=[]  SumOutDataTypeStr=single  SumOutMin=[]  SumOutMax=[]  SaturationOutDataTypeStr=single  SaturationOutMin=[]  SaturationOutMax=[]  PParamDataTypeStr=single  PParamMin=[]  PParamMax=[]  IParamDataTypeStr=single  IParamMin=[]  IParamMax=[]  DParamMin=[]  DParamMax=[]  NParamMin=[]  NParamMax=[]  KbParamDataTypeStr=single  KbParamMin=[]  KbParamMax=[]  KtParamMin=[]  KtParamMax=[]  KbOutDataTypeStr=single  KbOutMin=[]  KbOutMax=[]  KtOutMin=[]  KtOutMax=[]  IntegratorOutDataTypeStr=single  IntegratorOutMin=[]  IntegratorOutMax=[]  FilterOutMin=[]  FilterOutMax=[]  SumI1OutDataTypeStr=single  SumI1OutMin=[]  SumI1OutMax=[]  SumI2OutDataTypeStr=single  SumI2OutMin=[]  SumI2OutMax=[]  SumI3OutMin=[]  SumI3OutMax=[]  SumI4OutMin=[]  SumI4OutMax=[]  SumDOutMin=[]  SumDOutMax=[]  SumAccumDataTypeStr=single  SumI1AccumDataTypeStr=single  SumI2AccumDataTypeStr=single  DifferentiatorOutMin=[]  DifferentiatorOutMax=[]  FilterDiffOutCoefMin=[]  FilterDiffOutCoefMax=[]  ReciprocalOutMin=[]  ReciprocalOutMax=[]  SumDenOutMin=[]  SumDenOutMax=[]  SumNumOutMin=[]  SumNumOutMax=[]  DivideOutMin=[]  DivideOutMax=[]  UdiffTsProdOutMin=[]  UdiffTsProdOutMax=[]  NTsProdOutMin=[]  NTsProdOutMax=[]  UintegralTsProdOutMin=[]  UintegralTsProdOutMax=[]  UngainTsProdOutMin=[]  UngainTsProdOutMax=[]  ClampingZeroOutDataTypeStr=Inherit: Inherit via back propagation  ClampingZeroOutMin=[]  ClampingZeroOutMax=[]  FilterDenConstantOutDataTypeStr=Inherit: Inherit via back propagation  FilterDenConstantOutMin=[]  FilterDenConstantOutMax=[]  PCopyOutDataTypeStr=Inherit: Inherit via back propagation  PCopyOutMin=[]  PCopyOutMax=[]  NCopyOutDataTypeStr=Inherit: Inherit via back propagation  NCopyOutMin=[]  NCopyOutMax=[]  IntegratorContinuousStateAttributes=''  IntegratorStateIdentifier=di  IntegratorStateMustResolveToSignalObject=off  IntegratorRTWStateStorageClass=Auto  FilterContinuousStateAttributes=''  FilterStateMustResolveToSignalObject=off  FilterRTWStateStorageClass=Auto  ParallelPVariant=InternalParameters  IdealPVariant=Disabled  IVariant=InternalParameters  DVariant=Disabled  IntegratorVariant=Discrete  SatVariant=Enabled  AWVariant=BackCalculation  PCopyVariant=Disabled  TRVariant=Disabled  FdbkBlocksVariant=Forward  IdealPFdbkVariant=Disabled  SatFdbkVariant=Disabled  DerivativeFilterVariant=Disabled  NVariant=Disabled  NCopyVariant=Disabled_SignalSpec  FilterICVariant=Disabled  IntegratorICVariant=InternalICs  ExternalResetVariant=Disabled  TRSumVariant=Passthrough  SumFdbkVariant=Disabled  SumVariant=Sum_PI  TsampFilterVariant=InternalTs  TsampNgainVariant=Passthrough  TsampIntegralVariant=Passthrough  ExternalSaturationOutDataTypeStr=Inherit: Same as second input
  d Controller1 : slpidlib/PID Controller  Commented=on  Controller=PI  Form=Parallel  TimeDomain=Discrete-time  UseExternalTs=off  SampleTime=-1  IntegratorMethod=Forward Euler  FilterMethod=Forward Euler  ControllerParametersSource=internal  P=D_PI_P  I=D_PI_I  UseKiTs=off  D=0.09  N=100  UseFilter=on  TunerSelectOption=Transfer Function Based (PID Tuner App)  InitialConditionSource=internal  InitialConditionForIntegrator=0  InitialConditionForFilter=0  DifferentiatorICPrevScaledInput=0  ExternalReset=none  TrackingMode=off  Kt=1  LimitOutput=on  SatLimitsSource=internal  UpperSaturationLimit=D_PI_UP_LIMIT  LowerSaturationLimit=D_PI_LOW_LIMIT  LinearizeAsGain=off  AntiWindupMode=back-calculation  Kb=D_PI_KB  LimitIntegrator=off  UpperIntegratorSaturationLimit=inf  LowerIntegratorSaturationLimit=-inf  PGainOutDataTypeStr=single  PProdOutDataTypeStr=single  POutMin=[]  POutMax=[]  IGainOutDataTypeStr=single  IProdOutDataTypeStr=single  IOutMin=[]  IOutMax=[]  DOutMin=[]  DOutMax=[]  NOutMin=[]  NOutMax=[]  SumOutDataTypeStr=single  SumOutMin=[]  SumOutMax=[]  SaturationOutDataTypeStr=single  SaturationOutMin=[]  SaturationOutMax=[]  PParamDataTypeStr=single  PParamMin=[]  PParamMax=[]  IParamDataTypeStr=single  IParamMin=[]  IParamMax=[]  DParamMin=[]  DParamMax=[]  NParamMin=[]  NParamMax=[]  KbParamDataTypeStr=single  KbParamMin=[]  KbParamMax=[]  KtParamMin=[]  KtParamMax=[]  KbOutDataTypeStr=single  KbOutMin=[]  KbOutMax=[]  KtOutMin=[]  KtOutMax=[]  IntegratorOutDataTypeStr=single  IntegratorOutMin=[]  IntegratorOutMax=[]  FilterOutMin=[]  FilterOutMax=[]  SumI1OutDataTypeStr=single  SumI1OutMin=[]  SumI1OutMax=[]  SumI2OutDataTypeStr=single  SumI2OutMin=[]  SumI2OutMax=[]  SumI3OutMin=[]  SumI3OutMax=[]  SumI4OutMin=[]  SumI4OutMax=[]  SumDOutMin=[]  SumDOutMax=[]  SumAccumDataTypeStr=single  SumI1AccumDataTypeStr=single  SumI2AccumDataTypeStr=single  DifferentiatorOutMin=[]  DifferentiatorOutMax=[]  FilterDiffOutCoefMin=[]  FilterDiffOutCoefMax=[]  ReciprocalOutMin=[]  ReciprocalOutMax=[]  SumDenOutMin=[]  SumDenOutMax=[]  SumNumOutMin=[]  SumNumOutMax=[]  DivideOutMin=[]  DivideOutMax=[]  UdiffTsProdOutMin=[]  UdiffTsProdOutMax=[]  NTsProdOutMin=[]  NTsProdOutMax=[]  UintegralTsProdOutMin=[]  UintegralTsProdOutMax=[]  UngainTsProdOutMin=[]  UngainTsProdOutMax=[]  ClampingZeroOutDataTypeStr=Inherit: Inherit via back propagation  ClampingZeroOutMin=[]  ClampingZeroOutMax=[]  FilterDenConstantOutDataTypeStr=Inherit: Inherit via back propagation  FilterDenConstantOutMin=[]  FilterDenConstantOutMax=[]  PCopyOutDataTypeStr=Inherit: Inherit via back propagation  PCopyOutMin=[]  PCopyOutMax=[]  NCopyOutDataTypeStr=Inherit: Inherit via back propagation  NCopyOutMin=[]  NCopyOutMax=[]  IntegratorContinuousStateAttributes=''  IntegratorStateIdentifier=di  IntegratorStateMustResolveToSignalObject=off  IntegratorRTWStateStorageClass=Auto  FilterContinuousStateAttributes=''  FilterStateMustResolveToSignalObject=off  FilterRTWStateStorageClass=Auto  ParallelPVariant=InternalParameters  IdealPVariant=Disabled  IVariant=InternalParameters  DVariant=Disabled  IntegratorVariant=Discrete  SatVariant=Enabled  AWVariant=BackCalculation  PCopyVariant=Disabled  TRVariant=Disabled  FdbkBlocksVariant=Forward  IdealPFdbkVariant=Disabled  SatFdbkVariant=Disabled  DerivativeFilterVariant=Disabled  NVariant=Disabled  NCopyVariant=Disabled_SignalSpec  FilterICVariant=Disabled  IntegratorICVariant=InternalICs  ExternalResetVariant=Disabled  TRSumVariant=Passthrough  SumFdbkVariant=Disabled  SumVariant=Sum_PI  TsampFilterVariant=InternalTs  TsampNgainVariant=Passthrough  TsampIntegralVariant=Passthrough  ExternalSaturationOutDataTypeStr=Inherit: Same as second input
  id_back : Sum  Inputs=|++
  id_sum : Sum  Inputs=|+-
  iq_back : Sum  Inputs=|++
  iq_sum : Sum  Inputs=|+-
  park : Subsystem
  q Controller : slpidlib/PID Controller  Controller=PI  Form=Parallel  TimeDomain=Discrete-time  UseExternalTs=off  SampleTime=-1  IntegratorMethod=Forward Euler  FilterMethod=Forward Euler  ControllerParametersSource=internal  P=Q_PI_P  I=Q_PI_I  UseKiTs=off  D=0.09  N=100  UseFilter=on  TunerSelectOption=Transfer Function Based (PID Tuner App)  InitialConditionSource=internal  InitialConditionForIntegrator=0  InitialConditionForFilter=0  DifferentiatorICPrevScaledInput=0  ExternalReset=none  TrackingMode=off  Kt=1  LimitOutput=on  SatLimitsSource=internal  UpperSaturationLimit=Q_PI_UP_LIMIT  LowerSaturationLimit=Q_PI_LOW_LIMIT  LinearizeAsGain=off  AntiWindupMode=back-calculation  Kb=Q_PI_KB  LimitIntegrator=off  UpperIntegratorSaturationLimit=inf  LowerIntegratorSaturationLimit=-inf  PGainOutDataTypeStr=single  PProdOutDataTypeStr=single  POutMin=[]  POutMax=[]  IGainOutDataTypeStr=single  IProdOutDataTypeStr=single  IOutMin=[]  IOutMax=[]  DOutMin=[]  DOutMax=[]  NOutMin=[]  NOutMax=[]  SumOutDataTypeStr=single  SumOutMin=[]  SumOutMax=[]  SaturationOutDataTypeStr=single  SaturationOutMin=[]  SaturationOutMax=[]  PParamDataTypeStr=single  PParamMin=[]  PParamMax=[]  IParamDataTypeStr=single  IParamMin=[]  IParamMax=[]  DParamMin=[]  DParamMax=[]  NParamMin=[]  NParamMax=[]  KbParamDataTypeStr=single  KbParamMin=[]  KbParamMax=[]  KtParamMin=[]  KtParamMax=[]  KbOutDataTypeStr=single  KbOutMin=[]  KbOutMax=[]  KtOutMin=[]  KtOutMax=[]  IntegratorOutDataTypeStr=single  IntegratorOutMin=[]  IntegratorOutMax=[]  FilterOutMin=[]  FilterOutMax=[]  SumI1OutDataTypeStr=single  SumI1OutMin=[]  SumI1OutMax=[]  SumI2OutDataTypeStr=single  SumI2OutMin=[]  SumI2OutMax=[]  SumI3OutMin=[]  SumI3OutMax=[]  SumI4OutMin=[]  SumI4OutMax=[]  SumDOutMin=[]  SumDOutMax=[]  SumAccumDataTypeStr=single  SumI1AccumDataTypeStr=single  SumI2AccumDataTypeStr=single  DifferentiatorOutMin=[]  DifferentiatorOutMax=[]  FilterDiffOutCoefMin=[]  FilterDiffOutCoefMax=[]  ReciprocalOutMin=[]  ReciprocalOutMax=[]  SumDenOutMin=[]  SumDenOutMax=[]  SumNumOutMin=[]  SumNumOutMax=[]  DivideOutMin=[]  DivideOutMax=[]  UdiffTsProdOutMin=[]  UdiffTsProdOutMax=[]  NTsProdOutMin=[]  NTsProdOutMax=[]  UintegralTsProdOutMin=[]  UintegralTsProdOutMax=[]  UngainTsProdOutMin=[]  UngainTsProdOutMax=[]  ClampingZeroOutDataTypeStr=Inherit: Inherit via back propagation  ClampingZeroOutMin=[]  ClampingZeroOutMax=[]  FilterDenConstantOutDataTypeStr=Inherit: Inherit via back propagation  FilterDenConstantOutMin=[]  FilterDenConstantOutMax=[]  PCopyOutDataTypeStr=Inherit: Inherit via back propagation  PCopyOutMin=[]  PCopyOutMax=[]  NCopyOutDataTypeStr=Inherit: Inherit via back propagation  NCopyOutMin=[]  NCopyOutMax=[]  IntegratorContinuousStateAttributes=''  IntegratorStateIdentifier=qi  IntegratorStateMustResolveToSignalObject=off  IntegratorRTWStateStorageClass=Auto  FilterContinuousStateAttributes=''  FilterStateMustResolveToSignalObject=off  FilterRTWStateStorageClass=Auto  ParallelPVariant=InternalParameters  IdealPVariant=Disabled  IVariant=InternalParameters  DVariant=Disabled  IntegratorVariant=Discrete  SatVariant=Enabled  AWVariant=BackCalculation  PCopyVariant=Disabled  TRVariant=Disabled  FdbkBlocksVariant=Forward  IdealPFdbkVariant=Disabled  SatFdbkVariant=Disabled  DerivativeFilterVariant=Disabled  NVariant=Disabled  NCopyVariant=Disabled_SignalSpec  FilterICVariant=Disabled  IntegratorICVariant=InternalICs  ExternalResetVariant=Disabled  TRSumVariant=Passthrough  SumFdbkVariant=Disabled  SumVariant=Sum_PI  TsampFilterVariant=InternalTs  TsampNgainVariant=Passthrough  TsampIntegralVariant=Passthrough  ExternalSaturationOutDataTypeStr=Inherit: Same as second input
  q Controller1 : slpidlib/PID Controller  Commented=on  Controller=PI  Form=Parallel  TimeDomain=Discrete-time  UseExternalTs=off  SampleTime=-1  IntegratorMethod=Forward Euler  FilterMethod=Forward Euler  ControllerParametersSource=internal  P=Q_PI_P  I=Q_PI_I  UseKiTs=off  D=0.09  N=100  UseFilter=on  TunerSelectOption=Transfer Function Based (PID Tuner App)  InitialConditionSource=internal  InitialConditionForIntegrator=0  InitialConditionForFilter=0  DifferentiatorICPrevScaledInput=0  ExternalReset=none  TrackingMode=off  Kt=1  LimitOutput=on  SatLimitsSource=internal  UpperSaturationLimit=Q_PI_UP_LIMIT  LowerSaturationLimit=Q_PI_LOW_LIMIT  LinearizeAsGain=off  AntiWindupMode=back-calculation  Kb=Q_PI_KB  LimitIntegrator=off  UpperIntegratorSaturationLimit=inf  LowerIntegratorSaturationLimit=-inf  PGainOutDataTypeStr=single  PProdOutDataTypeStr=single  POutMin=[]  POutMax=[]  IGainOutDataTypeStr=single  IProdOutDataTypeStr=single  IOutMin=[]  IOutMax=[]  DOutMin=[]  DOutMax=[]  NOutMin=[]  NOutMax=[]  SumOutDataTypeStr=single  SumOutMin=[]  SumOutMax=[]  SaturationOutDataTypeStr=single  SaturationOutMin=[]  SaturationOutMax=[]  PParamDataTypeStr=single  PParamMin=[]  PParamMax=[]  IParamDataTypeStr=single  IParamMin=[]  IParamMax=[]  DParamMin=[]  DParamMax=[]  NParamMin=[]  NParamMax=[]  KbParamDataTypeStr=single  KbParamMin=[]  KbParamMax=[]  KtParamMin=[]  KtParamMax=[]  KbOutDataTypeStr=single  KbOutMin=[]  KbOutMax=[]  KtOutMin=[]  KtOutMax=[]  IntegratorOutDataTypeStr=single  IntegratorOutMin=[]  IntegratorOutMax=[]  FilterOutMin=[]  FilterOutMax=[]  SumI1OutDataTypeStr=single  SumI1OutMin=[]  SumI1OutMax=[]  SumI2OutDataTypeStr=single  SumI2OutMin=[]  SumI2OutMax=[]  SumI3OutMin=[]  SumI3OutMax=[]  SumI4OutMin=[]  SumI4OutMax=[]  SumDOutMin=[]  SumDOutMax=[]  SumAccumDataTypeStr=single  SumI1AccumDataTypeStr=single  SumI2AccumDataTypeStr=single  DifferentiatorOutMin=[]  DifferentiatorOutMax=[]  FilterDiffOutCoefMin=[]  FilterDiffOutCoefMax=[]  ReciprocalOutMin=[]  ReciprocalOutMax=[]  SumDenOutMin=[]  SumDenOutMax=[]  SumNumOutMin=[]  SumNumOutMax=[]  DivideOutMin=[]  DivideOutMax=[]  UdiffTsProdOutMin=[]  UdiffTsProdOutMax=[]  NTsProdOutMin=[]  NTsProdOutMax=[]  UintegralTsProdOutMin=[]  UintegralTsProdOutMax=[]  UngainTsProdOutMin=[]  UngainTsProdOutMax=[]  ClampingZeroOutDataTypeStr=Inherit: Inherit via back propagation  ClampingZeroOutMin=[]  ClampingZeroOutMax=[]  FilterDenConstantOutDataTypeStr=Inherit: Inherit via back propagation  FilterDenConstantOutMin=[]  FilterDenConstantOutMax=[]  PCopyOutDataTypeStr=Inherit: Inherit via back propagation  PCopyOutMin=[]  PCopyOutMax=[]  NCopyOutDataTypeStr=Inherit: Inherit via back propagation  NCopyOutMin=[]  NCopyOutMax=[]  IntegratorContinuousStateAttributes=''  IntegratorStateIdentifier=qi  IntegratorStateMustResolveToSignalObject=off  IntegratorRTWStateStorageClass=Auto  FilterContinuousStateAttributes=''  FilterStateMustResolveToSignalObject=off  FilterRTWStateStorageClass=Auto  ParallelPVariant=InternalParameters  IdealPVariant=Disabled  IVariant=InternalParameters  DVariant=Disabled  IntegratorVariant=Discrete  SatVariant=Enabled  AWVariant=BackCalculation  PCopyVariant=Disabled  TRVariant=Disabled  FdbkBlocksVariant=Forward  IdealPFdbkVariant=Disabled  SatFdbkVariant=Disabled  DerivativeFilterVariant=Disabled  NVariant=Disabled  NCopyVariant=Disabled_SignalSpec  FilterICVariant=Disabled  IntegratorICVariant=InternalICs  ExternalResetVariant=Disabled  TRSumVariant=Passthrough  SumFdbkVariant=Disabled  SumVariant=Sum_PI  TsampFilterVariant=InternalTs  TsampNgainVariant=Passthrough  TsampIntegralVariant=Passthrough  ExternalSaturationOutDataTypeStr=Inherit: Same as second input
  svpwm : Subsystem
  Tcm1 : Outport
  Tcm2 : Outport  Port=2
  Tcm3 : Outport  Port=3
  Id : Outport  Port=4
  Iq : Outport  Port=5
  Out1 : Outport  Port=6
  Out2 : Outport  Port=7
  Speed : Outport  Port=8
  Angle : Outport  Port=9
  wires:
  Theta/1 -> anti_park/3(theta), park/3(theta)
  Udc/1 -> svpwm/4(Udc)
  Tpwm/1 -> svpwm/3(Tpwm)
  svpwm/3(Tcm3) -> Tcm3/1
  svpwm/1(Tcm1) -> Tcm1/1
  svpwm/2(Tcm2) -> Tcm2/1
  Ia/1 -> clarke/1(Ia)
  Ib/1 -> clarke/2(Ib)
  Ic/1 -> clarke/3(Ic)
  park/1(Id) -> Id/1, MATLAB Function3/2(Id), id_sum/2
  park/2(Iq) -> Iq/1, MATLAB Function2/2(Iq), iq_sum/2
  Iq_ref/1 -> iq_sum/1
  iq_sum/1 -> q Controller/1
  we/1 -> MATLAB Function3/1(We), MATLAB Function2/1(We)
  q Controller/1 -> iq_back/1
  Id_ref/1 -> id_sum/1
  id_sum/1 -> d Controller/1
  d Controller/1 -> id_back/1
  Ls/1 -> EKF/6
  anti_park/2(Vbeta) -> EKF/2, svpwm/2(Ubeta)
  flux/1 -> EKF/7
  clarke/1(Ialpha) -> EKF/3, park/1(Ialpha)
  Rs/1 -> EKF/5
  anti_park/1(Valpha) -> EKF/1, svpwm/1(Ualpha)
  clarke/2(Ibeta) -> EKF/4, park/2(Ibeta)
  id_back/1 -> anti_park/1(Vd)
  iq_back/1 -> anti_park/2(Vq)
  ? -> S-Function Builder/1
  EKF/1 -> Out1/1
  EKF/2 -> Out2/1
  EKF/3 -> Speed/1
  EKF/4 -> Angle/1
